simulink library "WECSim_Lib_PTOs"  (R2020b)
settings: Solver=VariableStepAuto  StartTime=0.0  StopTime=10.0  RelTol=1e-3
undefined symbols (not defined in the file or in its folder): constraint, pto, simu, X, Y, Z
libraries: nesl_utility x71, sm_lib x46, WECSim_Lib_Body_Elements x1
(part 1 of 3)
settings Model: Creator=kmruehl  LastModifiedBy=akeeste

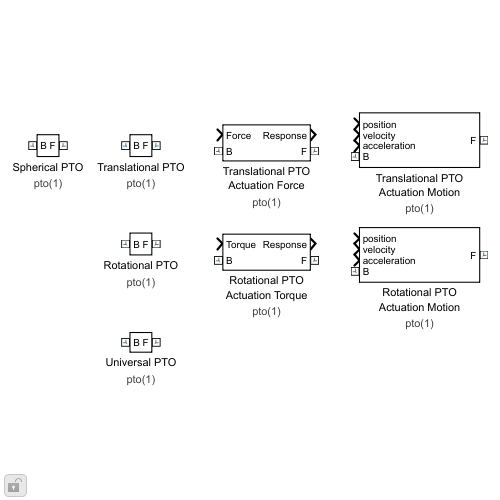
[thumbnail: Simulink's stored preview of the top-level diagram]
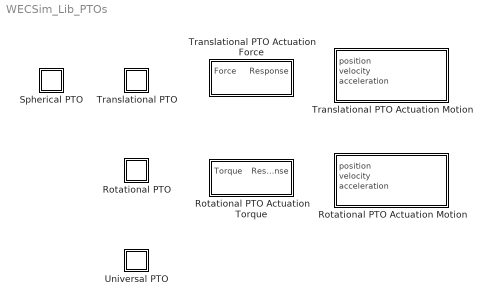
== system WECSim_Lib_PTOs ==
  Rotational PTO : Subsystem  mask(PTO){pto=pto(1)}
      mask prompts: pto "PTO Name:"
      mask help:
      | Constrains the follower to rotational motion relative to the base, about
      | the PTO's Y-direction and adds PTO stiffness and damping.
      |
      | The variable name input below must be 'pto(i)' where i=1,2,...
      | pto(i) must be defined in the input file with the following fields:
      |
      |     .name (required)
      |             String.
      |             PTO name. Must comply with Matlab's variable naming rules.
      |     .location (required)
      |             3x1 vector [x y z] in meters.
      |             PTO location. Default = [0 0 0]
      |     .stiffness (optional)
      |             Float.
      |             PTO linear spring stiffness. Default = 0
      |     .damping (optional)
      |             Float.
      |             PTO linear damping coefficient. Default = 0
      |     .orientation.z (optional)
      |             3x1 vector [x y z].
      |             Direction of the PTO's Z-coordinate. Default = [0 0 1]
      |     .orientation.y (optional)
      |             3x1 vector [x y z].
      |             Direction of the PTO's Y-coordinate. Default = [0 1 0]
      mask init:
      | if exist('pto','var')
      |     h=[gcb '/To Workspace'];
      |     responseName=['pto' num2str(pto.number) '_out'];
      |     set_param(h,'VariableName',responseName);
      |     h=[gcb '/Pitch PCC ' newline '(Revolute Joint)'];
      |     try % this should catch any version issue for which these parameters do not exist
      |         set_param(h,'upperLimitSpecify',pto.hardStops.upperLimitSpecify)
      |         set_param(h,'lowerLimitSpecify',pto.hardStops.lowerLimitSpecify)
      |     end
      |     if pto.extension.PositionTargetSpecify == 1
      |         set_param(h,'PositionTargetSpecify','on')
      |     else
      |         set_param(h,'PositionTargetSpecify','off')
      |     end
      | end
      | 
      | pto.checkLoc('E');
      settings: AttributesFormatString=%<pto>
      mask Help:
      | Constrains the follower to rotational motion relative to the base, about
      | the PTO's Y-direction and adds PTO stiffness and damping.
      | 
      | The variable name input below must be 'pto(i)' where i=1,2,...
      | pto(i) must be defined in the input file with the following fields:
      | 
      |     .name (required)
      |             String.
      |             PTO name. Must comply with Matlab's variable naming rules.
      |     .location (required)
      |             3x1 vector [x y z] in meters.
      |             PTO location. Default = [0 0 0]
      |     .stiffness (optional)
      |             Float.
      |             PTO linear spring stiffness. Default = 0
      |     .damping (optional)
      |             Float.
      |             PTO linear damping coefficient. Default = 0
      |     .orientation.z (optional)
      |             3x1 vector [x y z].
      |             Direction of the PTO's Z-coordinate. Default = [0 0 1]
      |     .orientation.y (optional)
      |             3x1 vector [x y z].
      |             Direction of the PTO's Y-coordinate. Default = [0 1 0]
  Rotational PTO Actuation Motion : Subsystem  mask(PTO){pto=pto(1)}
      mask prompts: pto "PTO Name:"
      mask help:
      | Constrains the follower to rotational motion relative to the base, about
      | the PTO's Y-direction and adds PTO stiffness and damping. Also enforces a
      | user-defined prescribed motion.
      |
      |
      | The variable name input below must be 'pto(i)' where i=1,2,...
      | pto(i) must be defined in the input file with the following fields:
      |
      |     .name (required)
      |             String.
      |             PTO name. Must comply with Matlab's variable naming rules.
      |     .location (required)
      |             3x1 vector [x y z] in meters.
      |             PTO location. Default = [0 0 0]
      |     .stiffness (optional)
      |             Float.
      |             PTO linear spring stiffness. Default = 0
      |     .damping (optional)
      |             Float.
      |             PTO linear damping coefficient. Default = 0
      |     .orientation.z (optional)
      |             3x1 vector [x y z].
      |             Direction of the PTO's Z-coordinate. Default = [0 0 1]
      |     .orientation.y (optional)
      |             3x1 vector [x y z].
      |             Direction of the PTO's Y-coordinate. Default = [0 1 0]
      mask init:
      | if exist('pto','var')
      |     h=[gcb '/To Workspace'];
      |     responseName=['pto' num2str(pto.number) '_out'];
      |     set_param(h,'VariableName',responseName);
      |     h=[gcb '/Pitch PCC ' newline '(Revolute Joint)'];
      |     try % this should catch any version issue for which these parameters do not exist
      |         set_param(h,'upperLimitSpecify',pto.hardStops.upperLimitSpecify)
      |         set_param(h,'lowerLimitSpecify',pto.hardStops.lowerLimitSpecify)
      |     end
      | end
      | 
      | pto.checkLoc('E');
      settings: AttributesFormatString=%<pto>
      mask Help:
      | Constrains the follower to rotational motion relative to the base, about
      | the PTO's Y-direction and adds PTO stiffness and damping. Also enforces a
      | user-defined prescribed motion.
      | 
      | 
      | The variable name input below must be 'pto(i)' where i=1,2,...
      | pto(i) must be defined in the input file with the following fields:
      | 
      |     .name (required)
      |             String.
      |             PTO name. Must comply with Matlab's variable naming rules.
      |     .location (required)
      |             3x1 vector [x y z] in meters.
      |             PTO location. Default = [0 0 0]
      |     .stiffness (optional)
      |             Float.
      |             PTO linear spring stiffness. Default = 0
      |     .damping (optional)
      |             Float.
      |             PTO linear damping coefficient. Default = 0
      |     .orientation.z (optional)
      |             3x1 vector [x y z].
      |             Direction of the PTO's Z-coordinate. Default = [0 0 1]
      |     .orientation.y (optional)
      |             3x1 vector [x y z].
      |             Direction of the PTO's Y-coordinate. Default = [0 1 0]
  Rotational PTO Actuation Torque : Subsystem  mask(PTO){pto=pto(1)}
      mask prompts: pto "PTO Name:"
      mask help:
      | Constrains the follower to rotational motion relative to the base, about
      | the PTO's Y-direction and adds PTO stiffness and damping. Also applies a
      | user-defined torque and outputs extension, velocity and acceleration.
      |
      |
      | The variable name input below must be 'pto(i)' where i=1,2,...
      | pto(i) must be defined in the input file with the following fields:
      |
      |     .name (required)
      |             String.
      |             PTO name. Must comply with Matlab's variable naming rules.
      |     .location (required)
      |             3x1 vector [x y z] in meters.
      |             PTO location. Default = [0 0 0]
      |     .stiffness (optional)
      |             Float.
      |             PTO linear spring stiffness. Default = 0
      |     .damping (optional)
      |             Float.
      |             PTO linear damping coefficient. Default = 0
      |     .orientation.z (optional)
      |             3x1 vector [x y z].
      |             Direction of the PTO's Z-coordinate. Default = [0 0 1]
      |     .orientation.y (optional)
      |             3x1 vector [x y z].
      |             Direction of the PTO's Y-coordinate. Default = [0 1 0]
      mask init: same as WECSim_Lib_PTOs/Rotational PTO
      settings: AttributesFormatString=%<pto>
      mask Help:
      | Constrains the follower to rotational motion relative to the base, about
      | the PTO's Y-direction and adds PTO stiffness and damping. Also applies a
      | user-defined torque and outputs extension, velocity and acceleration.
      | 
      | 
      | The variable name input below must be 'pto(i)' where i=1,2,...
      | pto(i) must be defined in the input file with the following fields:
      | 
      |     .name (required)
      |             String.
      |             PTO name. Must comply with Matlab's variable naming rules.
      |     .location (required)
      |             3x1 vector [x y z] in meters.
      |             PTO location. Default = [0 0 0]
      |     .stiffness (optional)
      |             Float.
      |             PTO linear spring stiffness. Default = 0
      |     .damping (optional)
      |             Float.
      |             PTO linear damping coefficient. Default = 0
      |     .orientation.z (optional)
      |             3x1 vector [x y z].
      |             Direction of the PTO's Z-coordinate. Default = [0 0 1]
      |     .orientation.y (optional)
      |             3x1 vector [x y z].
      |             Direction of the PTO's Y-coordinate. Default = [0 1 0]
  Spherical PTO : Subsystem  mask(PTOs){pto=pto(1)}
      mask prompts: pto "PTO Name:"
      mask help:
      | Constrains the follower to rotational motion relative to the base, fixing in
      | X,Y,Z but allowing rotation about each axis and adds PTO stiffness and damping.
      |
      | The variable name input below must be 'pto(i)' where i=1,2,...
      | pto(i) must be defined in the input file with the following fields:
      |
      |     .name (required)
      |             String.
      |            Constraint name. Must comply with Matlab's variable naming rules.
      |     .location (optional)
      |             3x1 vector [x y z] in meters.
      |             Constraint location. Default = [0 0 0]
      |     .stiffness (optional)
      |             Float.
      |             PTO linear spring stiffness. Default = 0
      |     .damping (optional)
      |             Float.
      |             PTO linear damping coefficient. Default = 0
      |     .orientation.z (optional)
      |             3x1 vector [x y z].
      |             Direction of the constraint's Z-coordinate. Default = [0 0 1]
      |     .orientation.y (optional)
      |             3x1 vector [x y z].
      |             Direction of the constraint's Y-coordinate. Default = [0 1 0]
      mask init:
      | if exist('pto','var')
      |     h=[gcb '/To Workspace'];
      |     responseName=['pto' num2str(pto.number) '_out'];
      |     set_param(h,'VariableName',responseName);
      |     h=[gcb '/Spherical Joint)'];
      |     try % this should catch any version issue for which these parameters do not exist
      |         set_param(h,'upperLimitSpecify',pto.hardStops.upperLimitSpecify)
      |         set_param(h,'lowerLimitSpecify',pto.hardStops.lowerLimitSpecify)
      |     end
      | end
      | if pto.extension.PositionTargetSpecify == 1
      |     set_param(h,'PositionTargetSpecify','on')
      | else
      |     set_param(h,'PositionTargetSpecify','off')
      | end
      | pto.checkLoc('W');
      settings: AttributesFormatString=%<pto>
      mask Help:
      | Constrains the follower to rotational motion relative to the base, fixing in
      | X,Y,Z but allowing rotation about each axis and adds PTO stiffness and damping.
      | 
      | The variable name input below must be 'pto(i)' where i=1,2,...
      | pto(i) must be defined in the input file with the following fields:
      | 
      |     .name (required)
      |             String.
      |            Constraint name. Must comply with Matlab's variable naming rules.
      |     .location (optional)
      |             3x1 vector [x y z] in meters.
      |             Constraint location. Default = [0 0 0]
      |     .stiffness (optional)
      |             Float.
      |             PTO linear spring stiffness. Default = 0
      |     .damping (optional)
      |             Float.
      |             PTO linear damping coefficient. Default = 0
      |     .orientation.z (optional)
      |             3x1 vector [x y z].
      |             Direction of the constraint's Z-coordinate. Default = [0 0 1]
      |     .orientation.y (optional)
      |             3x1 vector [x y z].
      |             Direction of the constraint's Y-coordinate. Default = [0 1 0]
  Translational PTO : Subsystem  mask(PTO){pto=pto(1)}
      mask prompts: pto "PTO Name:"
      mask help:
      | Constrains the follower to translational motion relative to the base, in
      | the PTO's Z-direction and adds PTO stiffness and damping.
      |
      |
      | The variable name input below must be 'pto(i)' where i=1,2,...
      | pto(i) must be defined in the input file with the following fields:
      |
      |     .name (required)
      |             String.
      |             PTO name. Must comply with Matlab's variable naming rules.
      |     .location (optional)
      |             3x1 vector [x y z] in meters.
      |             PTO location. Default = [0 0 0]
      |     .stiffness (optional)
      |             Float.
      |             PTO linear spring stiffness. Default = 0
      |     .damping (optional)
      |             Float.
      |             PTO linear damping coefficient. Default = 0
      |     .orientation.z (optional)
      |             3x1 vector [x y z].
      |             Direction of the PTO's Z-coordinate. Default = [0 0 1]
      |     .orientation.y (optional)
      |             3x1 vector [x y z].
      |             Direction of the PTO's Y-coordinate. Default = [0 1 0]
      mask init:
      | if exist('pto','var')
      |     h=[gcb '/To Workspace'];
      |     responseName=['pto' num2str(pto.number) '_out'];
      |     set_param(h,'VariableName',responseName);
      |     h=[gcb '/Translational PCC' newline '(Prismatic Joint)'];
      |     try % this should catch any version issue for which these parameters do not exist
      |         set_param(h,'upperLimitSpecify',pto.hardStops.upperLimitSpecify)
      |         set_param(h,'lowerLimitSpecify',pto.hardStops.lowerLimitSpecify)
      |     end
      |     if pto.extension.PositionTargetSpecify == 1
      |         set_param(h,'PositionTargetSpecify','on')
      |     else
      |         set_param(h,'PositionTargetSpecify','off')
      |     end
      | end
      | 
      | pto.checkLoc('W');
      settings: AttributesFormatString=%<pto>
      mask Help:
      | Constrains the follower to translational motion relative to the base, in
      | the PTO's Z-direction and adds PTO stiffness and damping.
      | 
      | 
      | The variable name input below must be 'pto(i)' where i=1,2,...
      | pto(i) must be defined in the input file with the following fields:
      | 
      |     .name (required)
      |             String.
      |             PTO name. Must comply with Matlab's variable naming rules.
      |     .location (optional)
      |             3x1 vector [x y z] in meters.
      |             PTO location. Default = [0 0 0]
      |     .stiffness (optional)
      |             Float.
      |             PTO linear spring stiffness. Default = 0
      |     .damping (optional)
      |             Float.
      |             PTO linear damping coefficient. Default = 0
      |     .orientation.z (optional)
      |             3x1 vector [x y z].
      |             Direction of the PTO's Z-coordinate. Default = [0 0 1]
      |     .orientation.y (optional)
      |             3x1 vector [x y z].
      |             Direction of the PTO's Y-coordinate. Default = [0 1 0]
  Translational PTO Actuation Force : Subsystem  mask(PTO){pto=pto(1)}
      mask prompts: pto "PTO Name:"
      mask help:
      | Constrains the follower to translational motion relative to the base, in
      | the PTO's Z-direction and adds PTO stiffness and damping. Also applies a
      | user-defined force and outputs extension, velocity, and acceleration.
      |
      |
      | The variable name input below must be 'pto(i)' where i=1,2,...
      | pto(i) must be defined in the input file with the following fields:
      |
      |     .name (required)
      |             String.
      |             PTO name. Must comply with Matlab's variable naming rules.
      |     .location (optional)
      |             3x1 vector [x y z] in meters.
      |             PTO location. Default = [0 0 0]
      |     .stifness (optional)
      |             Float.
      |             PTO linear spring stiffness. Default = 0
      |     .damping (optional)
      |             Float.
      |             PTO linear damping coefficient. Default = 0
      |     .orientation.z (optional)
      |             3x1 vector [x y z].
      |             Direction of the PTO's Z-coordinate. Default = [0 0 1]
      |     .orientation.y (optional)
      |             3x1 vector [x y z].
      |             Direction of the PTO's Y-coordinate. Default = [0 1 0]
      mask init:
      | if exist('pto','var')
      |     h=[gcb '/To Workspace'];
      |     responseName=['pto' num2str(pto.number) '_out'];
      |     set_param(h,'VariableName',responseName);
      |         h=[gcb '/Translational PCC' newline '(Prismatic Joint)'];
      |     try % this should catch any version issue for which these parameters do not exist
      |         set_param(h,'upperLimitSpecify',pto.hardStops.upperLimitSpecify)
      |         set_param(h,'lowerLimitSpecify',pto.hardStops.lowerLimitSpecify)
      |     end
      |     if pto.extension.PositionTargetSpecify == 1
      |         set_param(h,'PositionTargetSpecify','on')
      |     else
      |         set_param(h,'PositionTargetSpecify','off')
      |     end
      | end
      | 
      | pto.checkLoc('W');
      settings: AttributesFormatString=%<pto>
      mask Help:
      | Constrains the follower to translational motion relative to the base, in
      | the PTO's Z-direction and adds PTO stiffness and damping. Also applies a
      | user-defined force and outputs extension, velocity, and acceleration.
      | 
      | 
      | The variable name input below must be 'pto(i)' where i=1,2,...
      | pto(i) must be defined in the input file with the following fields:
      | 
      |     .name (required)
      |             String.
      |             PTO name. Must comply with Matlab's variable naming rules.
      |     .location (optional)
      |             3x1 vector [x y z] in meters.
      |             PTO location. Default = [0 0 0]
      |     .stifness (optional)
      |             Float.
      |             PTO linear spring stiffness. Default = 0
      |     .damping (optional)
      |             Float.
      |             PTO linear damping coefficient. Default = 0
      |     .orientation.z (optional)
      |             3x1 vector [x y z].
      |             Direction of the PTO's Z-coordinate. Default = [0 0 1]
      |     .orientation.y (optional)
      |             3x1 vector [x y z].
      |             Direction of the PTO's Y-coordinate. Default = [0 1 0]
  Translational PTO Actuation Motion : Subsystem  mask(PTO){pto=pto(1)}
      mask prompts: pto "PTO Name:"
      mask help:
      | Constrains the follower to translational motion relative to the base, in
      | the PTO's Z-direction and adds PTO stiffness and damping. Also enforces a
      | user-defined prescribed motion.
      |
      |
      | The variable name input below must be 'pto(i)' where i=1,2,...
      | pto(i) must be defined in the input file with the following fields:
      |
      |     .name (required)
      |             String.
      |             PTO name. Must comply with Matlab's variable naming rules.
      |     .location (optional)
      |             3x1 vector [x y z] in meters.
      |             PTO location. Default = [0 0 0]
      |     .stiffness (optional)
      |             Float.
      |             PTO linear spring stiffness. Default = 0
      |     .damping (optional)
      |             Float.
      |             PTO linear damping coefficient. Default = 0
      |     .orientation.z (optional)
      |             3x1 vector [x y z].
      |             Direction of the PTO's Z-coordinate. Default = [0 0 1]
      |     .orientation.y (optional)
      |             3x1 vector [x y z].
      |             Direction of the PTO's Y-coordinate. Default = [0 1 0]
      mask init:
      | if exist('pto','var')
      |     h=[gcb '/To Workspace'];
      |     responseName=['pto' num2str(pto.number) '_out'];
      |     set_param(h,'VariableName',responseName);
      |     h=[gcb '/Translational PCC' newline '(Prismatic Joint)'];
      |     try % this should catch any version issue for which these parameters do not exist
      |         set_param(h,'upperLimitSpecify',pto.hardStops.upperLimitSpecify)
      |         set_param(h,'lowerLimitSpecify',pto.hardStops.lowerLimitSpecify)
      |     end
      | end
      | 
      | pto.checkLoc('W');
      settings: AttributesFormatString=%<pto>
      mask Help:
      | Constrains the follower to translational motion relative to the base, in
      | the PTO's Z-direction and adds PTO stiffness and damping. Also enforces a
      | user-defined prescribed motion.
      | 
      | 
      | The variable name input below must be 'pto(i)' where i=1,2,...
      | pto(i) must be defined in the input file with the following fields:
      | 
      |     .name (required)
      |             String.
      |             PTO name. Must comply with Matlab's variable naming rules.
      |     .location (optional)
      |             3x1 vector [x y z] in meters.
      |             PTO location. Default = [0 0 0]
      |     .stiffness (optional)
      |             Float.
      |             PTO linear spring stiffness. Default = 0
      |     .damping (optional)
      |             Float.
      |             PTO linear damping coefficient. Default = 0
      |     .orientation.z (optional)
      |             3x1 vector [x y z].
      |             Direction of the PTO's Z-coordinate. Default = [0 0 1]
      |     .orientation.y (optional)
      |             3x1 vector [x y z].
      |             Direction of the PTO's Y-coordinate. Default = [0 1 0]
  Universal PTO : Subsystem  mask(PTOs){pto=pto(1)}
      mask prompts: pto "PTO Name:"
      mask help:
      | Constrains the follower to rotational motion relative to the base, fixing in
      | X,Y,Z but allowing rotation about each axis and adds PTO stiffness and damping.
      |
      | The variable name input below must be 'pto(i)' where i=1,2,...
      | pto(i) must be defined in the input file with the following fields:
      |
      |     .name (required)
      |             String.
      |            Constraint name. Must comply with Matlab's variable naming rules.
      |     .location (optional)
      |             3x1 vector [x y z] in meters.
      |             Constraint location. Default = [0 0 0]
      |     .stiffness (optional)
      |             Float.
      |             PTO linear spring stiffness. Default = 0
      |     .damping (optional)
      |             Float.
      |             PTO linear damping coefficient. Default = 0
      |     .orientation.z (optional)
      |             3x1 vector [x y z].
      |             Direction of the constraint's Z-coordinate. Default = [0 0 1]
      |     .orientation.y (optional)
      |             3x1 vector [x y z].
      |             Direction of the constraint's Y-coordinate. Default = [0 1 0]
      mask init:
      | if exist('pto','var')
      |     h=[gcb '/To Workspace'];
      |     responseName=['pto' num2str(pto.number) '_out'];
      |     set_param(h,'VariableName',responseName);
      |     h=[gcb '/Universal Joint'];
      |     try % this should catch any version issue for which these parameters do not exist
      |         set_param(h,'RxUpperLimitSpecify',pto.hardStops.upperLimitSpecify(1))
      |         set_param(h,'RxLowerLimitSpecify',pto.hardStops.lowerLimitSpecify(1))
      |         set_param(h,'RyUpperLimitSpecify',pto.hardStops.upperLimitSpecify(2))
      |         set_param(h,'RyLowerLimitSpecify',pto.hardStops.lowerLimitSpecify(2))
      |     end
      | end
      | if pto.extension.PositionTargetSpecify == 1
      |     set_param(h,'RxPositionTargetSpecify','on')
      |     set_param(h,'RyPositionTargetSpecify','on')
      | else
      |     set_param(h,'RxPositionTargetSpecify','off')
      |     set_param(h,'RyPositionTargetSpecify','off')
      | end
      | pto.checkLoc('W');
      settings: AttributesFormatString=%<pto>
      mask Help:
      | Constrains the follower to rotational motion relative to the base, fixing in
      | X,Y,Z but allowing rotation about each axis and adds PTO stiffness and damping.
      | 
      | The variable name input below must be 'pto(i)' where i=1,2,...
      | pto(i) must be defined in the input file with the following fields:
      | 
      |     .name (required)
      |             String.
      |            Constraint name. Must comply with Matlab's variable naming rules.
      |     .location (optional)
      |             3x1 vector [x y z] in meters.
      |             Constraint location. Default = [0 0 0]
      |     .stiffness (optional)
      |             Float.
      |             PTO linear spring stiffness. Default = 0
      |     .damping (optional)
      |             Float.
      |             PTO linear damping coefficient. Default = 0
      |     .orientation.z (optional)
      |             3x1 vector [x y z].
      |             Direction of the constraint's Z-coordinate. Default = [0 0 1]
      |     .orientation.y (optional)
      |             3x1 vector [x y z].
      |             Direction of the constraint's Y-coordinate. Default = [0 1 0]

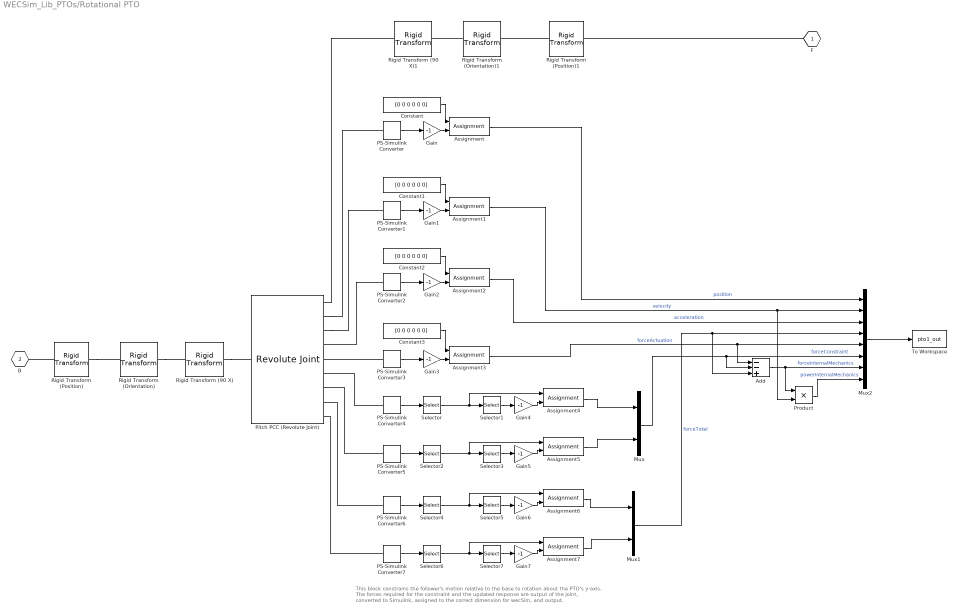
== system WECSim_Lib_PTOs/Rotational PTO ==
  note: This block constrains the follower's motion relative to the base to rotation about the PTO's y-axis. The forces required for the constraint and the updated response are output of the joint, converted to Simulink, assigned to the correct dimension for wecSim, and output.
  Add : Sum  Inputs=--+
  "Assignment " : Assignment  IndexOptions=Index vector (dialog)  Indices=5  OutputSizes=1
  Assignment1 : Assignment  IndexOptions=Index vector (dialog)  Indices=5  OutputSizes=1
  Assignment2 : Assignment  IndexOptions=Index vector (dialog)  Indices=5  OutputSizes=1
  Assignment3 : Assignment  IndexOptions=Index vector (dialog)  Indices=5  OutputSizes=1
  Assignment{4..7} (4 alike) : Assignment  DiagnosticForDimensions=Warning  IndexOptions=Index vector (dialog)  Indices=2  OutputSizes=1
  Constant{,1..3} (4 alike) : Constant  Value=[0 0 0 0 0 0]
  Gain{,1..7} (8 alike) : Gain  Gain=-1
  Mux : Mux  Inputs=2
  Mux1 : Mux  Inputs=2
  Mux2 : Mux  Inputs=8
  PS-Simulink Converter{,1..7} (8 alike) : nesl_utility/PS-Simulink Converter  PhysicalDomain=network_engine_domain  SubClassName=ps_output  LeftPortType=input  RightPortType=output  PseudoPeriodic=off  Frequencies=[]  VectorFormat=1-D array  Unit=1  AffineConversion=off
  Pitch PCC (Revolute Joint) : sm_lib/Joints/Revolute Joint  JointMode=Normal  CompositeWrenchDir=BaseOnFollower  CompositeWrenchFrame=BaseFrame  SenseConstraintForce=on  SenseConstraintTorque=on  SenseTotalForce=on  SenseTotalTorque=on  PositionTargetSpecify=off  PositionTargetPriority=High  PositionTargetValue=-pto.extension.PositionTargetValue  PositionTargetValueUnits=deg  VelocityTargetSpecify=off  VelocityTargetPriority=High  VelocityTargetValue=0  VelocityTargetValueUnits=deg/s  EquilibriumPosition=pto.equilibriumPosition  EquilibriumPositionUnits=deg  SpringStiffness=pto.stiffness  SpringStiffnessUnits=N*m/rad  DampingCoefficient=pto.damping  DampingCoefficientUnits=N*m/(rad/s)  LowerLimitSpecify=off  LowerLimitBound=pto.hardStops.lowerLimitBound  LowerLimitBoundUnits=deg  LowerLimitStiffness=pto.hardStops.lowerLimitStiffness  LowerLimitStiffnessUnits=N*m/deg  LowerLimitDamping=pto.hardStops.lowerLimitDamping  LowerLimitDampingUnits=N*m/(deg/s)  LowerLimitTransitionRegionWidth=pto.hardStops.lowerLimitTransitionRegionWidth  LowerLimitTransitionRegionWidthUnits=deg  UpperLimitSpecify=off  UpperLimitBound=pto.hardStops.upperLimitBound  UpperLimitBoundUnits=deg  UpperLimitStiffness=pto.hardStops.upperLimitStiffness  UpperLimitStiffnessUnits=N*m/deg  UpperLimitDamping=pto.hardStops.upperLimitDamping  UpperLimitDampingUnits=N*m/(deg/s)  UpperLimitTransitionRegionWidth=pto.hardStops.upperLimitTransitionRegionWidth  UpperLimitTransitionRegionWidthUnits=deg  TorqueActuationMode=NoTorque  MotionActuationMode=ComputedMotion  SensePosition=on  SenseVelocity=on  SenseAcceleration=on  SenseTorqueForce=on  SenseLowerLimitTorqueForce=off  SenseUpperLimitTorqueForce=off
  Product : Product
  Rigid Transform (Position) : sm_lib/Frames and Transforms/Rigid Transform  RotationMethod=None  FollAlignAxisA=+X  BaseAlignAxisA=+Y  FollAlignAxisB=+Y  BaseAlignAxisB=+Z  RotationStandardAxis=+Y  RotationAngle=0  RotationAngleUnits=rad  RotationArbitraryAxis=[0 1 0]  RotationSequenceAxes=FollowerAxes  RotationSequence=XYX  RotationSequenceAngles=[0 0 0]  RotationSequenceAnglesUnits=deg  RotationMatrix=[1 0 0; 0 1 0; 0 0 1]  Quaternion=[1 0 0 0]  TranslationMethod=Cartesian  TranslationCartesianOffset=pto.initial.displacement + pto.location  TranslationCartesianOffsetUnits=m  TranslationStandardAxis=+Z  TranslationStandardOffset=0  TranslationStandardOffsetUnits=m  TranslationROffset=0  TranslationROffsetUnits=m  TranslationThetaOffset=0  TranslationThetaOffsetUnits=deg  TranslationZOffset=0  TranslationZOffsetUnits=m
  Rigid Transform (Position)1 : sm_lib/Frames and Transforms/Rigid Transform  RotationMethod=None  FollAlignAxisA=+X  BaseAlignAxisA=+Y  FollAlignAxisB=+Y  BaseAlignAxisB=+Z  RotationStandardAxis=+Y  RotationAngle=0  RotationAngleUnits=rad  RotationArbitraryAxis=[0 1 0]  RotationSequenceAxes=FollowerAxes  RotationSequence=XYX  RotationSequenceAngles=[0 0 0]  RotationSequenceAnglesUnits=deg  RotationMatrix=[1 0 0; 0 1 0; 0 0 1]  Quaternion=[1 0 0 0]  TranslationMethod=Cartesian  TranslationCartesianOffset=pto.initial.displacement + pto.location  TranslationCartesianOffsetUnits=m  TranslationStandardAxis=+Z  TranslationStandardOffset=0  TranslationStandardOffsetUnits=m  TranslationROffset=0  TranslationROffsetUnits=m  TranslationThetaOffset=0  TranslationThetaOffsetUnits=deg  TranslationZOffset=0  TranslationZOffsetUnits=m
  Rigid Transform (90 X) : sm_lib/Frames and Transforms/Rigid Transform  RotationMethod=StandardAxis  FollAlignAxisA=+X  BaseAlignAxisA=+Y  FollAlignAxisB=+Y  BaseAlignAxisB=+Z  RotationStandardAxis=+X  RotationAngle=90  RotationAngleUnits=deg  RotationArbitraryAxis=[0 1 0]  RotationSequenceAxes=FollowerAxes  RotationSequence=XYX  RotationSequenceAngles=[0 0 0]  RotationSequenceAnglesUnits=deg  RotationMatrix=[1 0 0; 0 1 0; 0 0 1]  Quaternion=[1 0 0 0]  TranslationMethod=None  TranslationCartesianOffset=0  TranslationCartesianOffsetUnits=m  TranslationStandardAxis=+Z  TranslationStandardOffset=0  TranslationStandardOffsetUnits=m  TranslationROffset=0  TranslationROffsetUnits=m  TranslationThetaOffset=0  TranslationThetaOffsetUnits=deg  TranslationZOffset=0  TranslationZOffsetUnits=m
  Rigid Transform (90 X)1 : sm_lib/Frames and Transforms/Rigid Transform  RotationMethod=StandardAxis  FollAlignAxisA=+X  BaseAlignAxisA=+Y  FollAlignAxisB=+Y  BaseAlignAxisB=+Z  RotationStandardAxis=+X  RotationAngle=90  RotationAngleUnits=deg  RotationArbitraryAxis=[0 1 0]  RotationSequenceAxes=FollowerAxes  RotationSequence=XYX  RotationSequenceAngles=[0 0 0]  RotationSequenceAnglesUnits=deg  RotationMatrix=[1 0 0; 0 1 0; 0 0 1]  Quaternion=[1 0 0 0]  TranslationMethod=None  TranslationCartesianOffset=0  TranslationCartesianOffsetUnits=m  TranslationStandardAxis=+Z  TranslationStandardOffset=0  TranslationStandardOffsetUnits=m  TranslationROffset=0  TranslationROffsetUnits=m  TranslationThetaOffset=0  TranslationThetaOffsetUnits=deg  TranslationZOffset=0  TranslationZOffsetUnits=m
  Rigid Transform (Orientation) : sm_lib/Frames and Transforms/Rigid Transform  RotationMethod=RotationMatrix  FollAlignAxisA=+X  BaseAlignAxisA=+Y  FollAlignAxisB=+Y  BaseAlignAxisB=+Z  RotationStandardAxis=+Y  RotationAngle=0  RotationAngleUnits=rad  RotationArbitraryAxis=[0 1 0]  RotationSequenceAxes=FollowerAxes  RotationSequence=XYX  RotationSequenceAngles=[0 0 0]  RotationSequenceAnglesUnits=deg  RotationMatrix=pto.orientation.rotationMatrix  Quaternion=[1 0 0 0]  TranslationMethod=None  TranslationCartesianOffset=0  TranslationCartesianOffsetUnits=m  TranslationStandardAxis=+Z  TranslationStandardOffset=0  TranslationStandardOffsetUnits=m  TranslationROffset=0  TranslationROffsetUnits=m  TranslationThetaOffset=0  TranslationThetaOffsetUnits=deg  TranslationZOffset=0  TranslationZOffsetUnits=m
  Rigid Transform (Orientation)1 : sm_lib/Frames and Transforms/Rigid Transform  RotationMethod=RotationMatrix  FollAlignAxisA=+X  BaseAlignAxisA=+Y  FollAlignAxisB=+Y  BaseAlignAxisB=+Z  RotationStandardAxis=+Y  RotationAngle=0  RotationAngleUnits=rad  RotationArbitraryAxis=[0 1 0]  RotationSequenceAxes=FollowerAxes  RotationSequence=XYX  RotationSequenceAngles=[0 0 0]  RotationSequenceAnglesUnits=deg  RotationMatrix=pto.orientation.rotationMatrix  Quaternion=[1 0 0 0]  TranslationMethod=None  TranslationCartesianOffset=0  TranslationCartesianOffsetUnits=m  TranslationStandardAxis=+Z  TranslationStandardOffset=0  TranslationStandardOffsetUnits=m  TranslationROffset=0  TranslationROffsetUnits=m  TranslationThetaOffset=0  TranslationThetaOffsetUnits=deg  TranslationZOffset=0  TranslationZOffsetUnits=m
  Selector{,2,4,6} (4 alike) : Selector  InputPortWidth=3  IndexOptions=Index vector (dialog)  Indices=[1 3 2]  OutputSizes=1
  Selector{1,3,5,7} (4 alike) : Selector  InputPortWidth=3  IndexOptions=Index vector (dialog)  Indices=[2]  OutputSizes=1
  To Workspace : ToWorkspace  VariableName=pto1_out  SaveFormat=Structure With Time  SampleTime=simu.dtOut
  F : PMIOPort  Side=Right
  B : PMIOPort  Port=2  Side=Left
  wires:
  Assignment3/1 -> Add/1, Mux2/5  "forceActuation"
  Assignment2/1 -> Mux2/3  "acceleration"
  PS-Simulink Converter3/1 -> Gain3/1
  Gain3/1 -> Assignment3/2
  Constant3/1 -> Assignment3/1
  Gain2/1 -> Assignment2/2
  Constant2/1 -> Assignment2/1
  PS-Simulink Converter2/1 -> Gain2/1
  PS-Simulink Converter1/1 -> Gain1/1
  Gain1/1 -> Assignment1/2
  Constant1/1 -> Assignment1/1
  "Assignment "/1 -> Mux2/1  "position"
  Gain/1 -> "Assignment "/2
  PS-Simulink Converter/1 -> Gain/1
  Constant/1 -> "Assignment "/1
  Assignment6/1 -> Mux1/1
  Assignment7/1 -> Mux1/2
  PS-Simulink Converter7/1 -> Selector6/1
  PS-Simulink Converter6/1 -> Selector4/1
  Gain6/1 -> Assignment6/2
  Selector5/1 -> Gain6/1
  Selector4/1 -> Assignment6/1, Selector5/1
  Gain7/1 -> Assignment7/2
  Selector7/1 -> Gain7/1
  Selector6/1 -> Assignment7/1, Selector7/1
  Mux2/1 -> To Workspace/1
  PS-Simulink Converter4/1 -> Selector/1
  PS-Simulink Converter5/1 -> Selector2/1
  Assignment4/1 -> Mux/1
  Assignment5/1 -> Mux/2
  Gain4/1 -> Assignment4/2
  Selector1/1 -> Gain4/1
  Selector/1 -> Selector1/1, Assignment4/1
  Gain5/1 -> Assignment5/2
  Selector3/1 -> Gain5/1
  Selector2/1 -> Selector3/1, Assignment5/1
  Product/1 -> Mux2/8  "powerInternalMechanics"
  Assignment1/1 -> Product/2, Mux2/2  "velocity"
  Add/1 -> Mux2/7, Product/1  "forceInternalMechanics"
  Mux/1 -> Mux2/6, Add/2  "forceConstraint"
  Mux1/1 -> Add/3, Mux2/4  "forceTotal"
  connections:
  Rigid Transform (Position)/RConn1 -- Rigid Transform (Orientation)/LConn1
  Rigid Transform (Orientation)1/RConn1 -- Rigid Transform (90 X)1/LConn1
  Rigid Transform (Orientation)/RConn1 -- Rigid Transform (90 X)/LConn1
  Rigid Transform (Position)1/RConn1 -- Rigid Transform (Orientation)1/LConn1
  Rigid Transform (90 X)/RConn1 -- Pitch PCC (Revolute Joint)/LConn1
  F/RConn1 -- Rigid Transform (Position)1/LConn1
  Rigid Transform (90 X)1/RConn1 -- Pitch PCC (Revolute Joint)/RConn1
  PS-Simulink Converter3/LConn1 -- Pitch PCC (Revolute Joint)/RConn5
  PS-Simulink Converter2/LConn1 -- Pitch PCC (Revolute Joint)/RConn4
  Pitch PCC (Revolute Joint)/RConn3 -- PS-Simulink Converter1/LConn1
  Pitch PCC (Revolute Joint)/RConn2 -- PS-Simulink Converter/LConn1
  PS-Simulink Converter4/LConn1 -- Pitch PCC (Revolute Joint)/RConn6
  PS-Simulink Converter5/LConn1 -- Pitch PCC (Revolute Joint)/RConn7
  PS-Simulink Converter6/LConn1 -- Pitch PCC (Revolute Joint)/RConn8
  PS-Simulink Converter7/LConn1 -- Pitch PCC (Revolute Joint)/RConn9
  Rigid Transform (Position)/LConn1 -- B/RConn1

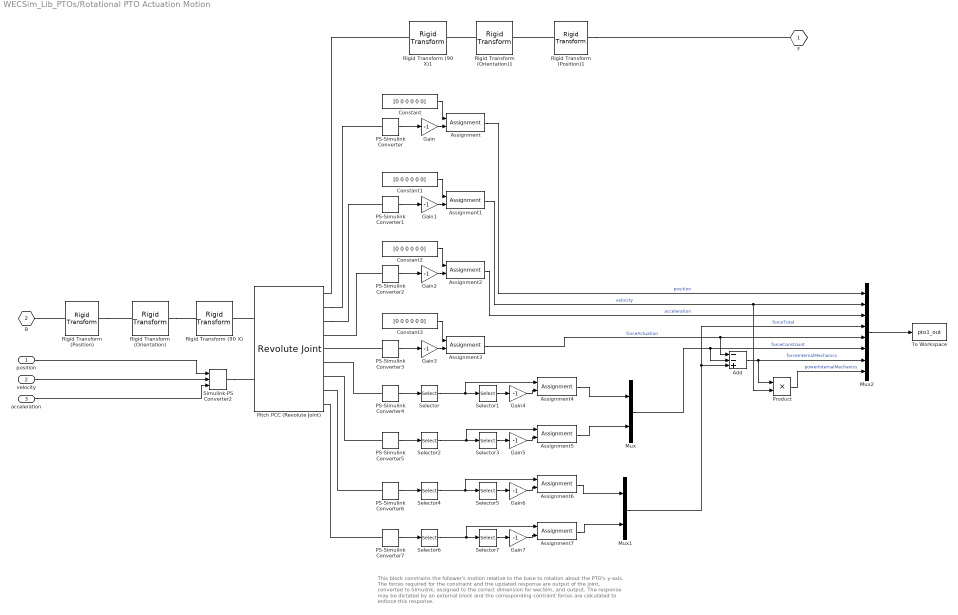
== system WECSim_Lib_PTOs/Rotational PTO Actuation Motion ==
  note: This block constrains the follower's motion relative to the base to rotation about the PTO's y-axis. The forces required for the constraint and the updated response are output of the joint, converted to Simulink, assigned to the correct dimension for wecSim, and output.
      |
      | The response may be dictated by an external block and the corresponding contraint forces are calculated to enforce this response.
  position : Inport
  velocity : Inport  Port=2
  acceleration : Inport  Port=3
  Add : Sum  Inputs=--+
  "Assignment " : Assignment  IndexOptions=Index vector (dialog)  Indices=5  OutputSizes=1
  Assignment1 : Assignment  IndexOptions=Index vector (dialog)  Indices=5  OutputSizes=1
  Assignment2 : Assignment  IndexOptions=Index vector (dialog)  Indices=5  OutputSizes=1
  Assignment3 : Assignment  IndexOptions=Index vector (dialog)  Indices=5  OutputSizes=1
  Assignment{4..7} (4 alike) : Assignment  DiagnosticForDimensions=Warning  IndexOptions=Index vector (dialog)  Indices=2  OutputSizes=1
  Constant{,1..3} (4 alike) : Constant  Value=[0 0 0 0 0 0]
  Gain{,1..7} (8 alike) : Gain  Gain=-1
  Mux : Mux  Inputs=2
  Mux1 : Mux  Inputs=2
  Mux2 : Mux  Inputs=8
  PS-Simulink Converter{,1..7} (8 alike) : nesl_utility/PS-Simulink Converter  PhysicalDomain=network_engine_domain  SubClassName=ps_output  LeftPortType=input  RightPortType=output  PseudoPeriodic=off  Frequencies=[]  VectorFormat=1-D array  Unit=1  AffineConversion=off
  Pitch PCC (Revolute Joint) : sm_lib/Joints/Revolute Joint  JointMode=Normal  CompositeWrenchDir=BaseOnFollower  CompositeWrenchFrame=BaseFrame  SenseConstraintForce=on  SenseConstraintTorque=on  SenseTotalForce=on  SenseTotalTorque=on  PositionTargetSpecify=off  PositionTargetPriority=High  PositionTargetValue=0  PositionTargetValueUnits=deg  VelocityTargetSpecify=off  VelocityTargetPriority=High  VelocityTargetValue=0  VelocityTargetValueUnits=deg/s  EquilibriumPosition=pto.equilibriumPosition  EquilibriumPositionUnits=deg  SpringStiffness=pto.stiffness  SpringStiffnessUnits=N*m/rad  DampingCoefficient=pto.damping  DampingCoefficientUnits=N*m/(rad/s)  LowerLimitSpecify=off  LowerLimitBound=pto.hardStops.lowerLimitBound  LowerLimitBoundUnits=deg  LowerLimitStiffness=pto.hardStops.lowerLimitStiffness  LowerLimitStiffnessUnits=N*m/deg  LowerLimitDamping=pto.hardStops.lowerLimitDamping  LowerLimitDampingUnits=N*m/(deg/s)  LowerLimitTransitionRegionWidth=pto.hardStops.lowerLimitTransitionRegionWidth  LowerLimitTransitionRegionWidthUnits=deg  UpperLimitSpecify=off  UpperLimitBound=pto.hardStops.upperLimitBound  UpperLimitBoundUnits=deg  UpperLimitStiffness=pto.hardStops.upperLimitStiffness  UpperLimitStiffnessUnits=N*m/deg  UpperLimitDamping=pto.hardStops.upperLimitDamping  UpperLimitDampingUnits=N*m/(deg/s)  UpperLimitTransitionRegionWidth=pto.hardStops.upperLimitTransitionRegionWidth  UpperLimitTransitionRegionWidthUnits=deg  TorqueActuationMode=ComputedTorque  MotionActuationMode=InputMotion  SensePosition=on  SenseVelocity=on  SenseAcceleration=on  SenseTorqueForce=on  SenseLowerLimitTorqueForce=off  SenseUpperLimitTorqueForce=off
  Product : Product
  Rigid Transform (Position) : sm_lib/Frames and Transforms/Rigid Transform  RotationMethod=None  FollAlignAxisA=+X  BaseAlignAxisA=+Y  FollAlignAxisB=+Y  BaseAlignAxisB=+Z  RotationStandardAxis=+Y  RotationAngle=0  RotationAngleUnits=rad  RotationArbitraryAxis=[0 1 0]  RotationSequenceAxes=FollowerAxes  RotationSequence=XYX  RotationSequenceAngles=[0 0 0]  RotationSequenceAnglesUnits=deg  RotationMatrix=[1 0 0; 0 1 0; 0 0 1]  Quaternion=[1 0 0 0]  TranslationMethod=Cartesian  TranslationCartesianOffset=pto.initial.displacement + pto.location  TranslationCartesianOffsetUnits=m  TranslationStandardAxis=+Z  TranslationStandardOffset=0  TranslationStandardOffsetUnits=m  TranslationROffset=0  TranslationROffsetUnits=m  TranslationThetaOffset=0  TranslationThetaOffsetUnits=deg  TranslationZOffset=0  TranslationZOffsetUnits=m
  Rigid Transform (Position)1 : sm_lib/Frames and Transforms/Rigid Transform  RotationMethod=None  FollAlignAxisA=+X  BaseAlignAxisA=+Y  FollAlignAxisB=+Y  BaseAlignAxisB=+Z  RotationStandardAxis=+Y  RotationAngle=0  RotationAngleUnits=rad  RotationArbitraryAxis=[0 1 0]  RotationSequenceAxes=FollowerAxes  RotationSequence=XYX  RotationSequenceAngles=[0 0 0]  RotationSequenceAnglesUnits=deg  RotationMatrix=[1 0 0; 0 1 0; 0 0 1]  Quaternion=[1 0 0 0]  TranslationMethod=Cartesian  TranslationCartesianOffset=pto.initial.displacement + pto.location  TranslationCartesianOffsetUnits=m  TranslationStandardAxis=+Z  TranslationStandardOffset=0  TranslationStandardOffsetUnits=m  TranslationROffset=0  TranslationROffsetUnits=m  TranslationThetaOffset=0  TranslationThetaOffsetUnits=deg  TranslationZOffset=0  TranslationZOffsetUnits=m
  Rigid Transform (90 X) : sm_lib/Frames and Transforms/Rigid Transform  RotationMethod=StandardAxis  FollAlignAxisA=+X  BaseAlignAxisA=+Y  FollAlignAxisB=+Y  BaseAlignAxisB=+Z  RotationStandardAxis=+X  RotationAngle=90  RotationAngleUnits=deg  RotationArbitraryAxis=[0 1 0]  RotationSequenceAxes=FollowerAxes  RotationSequence=XYX  RotationSequenceAngles=[0 0 0]  RotationSequenceAnglesUnits=deg  RotationMatrix=[1 0 0; 0 1 0; 0 0 1]  Quaternion=[1 0 0 0]  TranslationMethod=None  TranslationCartesianOffset=constraint.location  TranslationCartesianOffsetUnits=m  TranslationStandardAxis=+Z  TranslationStandardOffset=0  TranslationStandardOffsetUnits=m  TranslationROffset=0  TranslationROffsetUnits=m  TranslationThetaOffset=0  TranslationThetaOffsetUnits=deg  TranslationZOffset=0  TranslationZOffsetUnits=m
  Rigid Transform (90 X)1 : sm_lib/Frames and Transforms/Rigid Transform  RotationMethod=StandardAxis  FollAlignAxisA=+X  BaseAlignAxisA=+Y  FollAlignAxisB=+Y  BaseAlignAxisB=+Z  RotationStandardAxis=+X  RotationAngle=90  RotationAngleUnits=deg  RotationArbitraryAxis=[0 1 0]  RotationSequenceAxes=FollowerAxes  RotationSequence=XYX  RotationSequenceAngles=[0 0 0]  RotationSequenceAnglesUnits=deg  RotationMatrix=[1 0 0; 0 1 0; 0 0 1]  Quaternion=[1 0 0 0]  TranslationMethod=None  TranslationCartesianOffset=constraint.location  TranslationCartesianOffsetUnits=m  TranslationStandardAxis=+Z  TranslationStandardOffset=0  TranslationStandardOffsetUnits=m  TranslationROffset=0  TranslationROffsetUnits=m  TranslationThetaOffset=0  TranslationThetaOffsetUnits=deg  TranslationZOffset=0  TranslationZOffsetUnits=m
  Rigid Transform (Orientation) : sm_lib/Frames and Transforms/Rigid Transform  RotationMethod=RotationMatrix  FollAlignAxisA=+X  BaseAlignAxisA=+Y  FollAlignAxisB=+Y  BaseAlignAxisB=+Z  RotationStandardAxis=+Y  RotationAngle=0  RotationAngleUnits=rad  RotationArbitraryAxis=[0 1 0]  RotationSequenceAxes=FollowerAxes  RotationSequence=XYX  RotationSequenceAngles=[0 0 0]  RotationSequenceAnglesUnits=deg  RotationMatrix=pto.orientation.rotationMatrix  Quaternion=[1 0 0 0]  TranslationMethod=None  TranslationCartesianOffset=constraint.location  TranslationCartesianOffsetUnits=m  TranslationStandardAxis=+Z  TranslationStandardOffset=0  TranslationStandardOffsetUnits=m  TranslationROffset=0  TranslationROffsetUnits=m  TranslationThetaOffset=0  TranslationThetaOffsetUnits=deg  TranslationZOffset=0  TranslationZOffsetUnits=m
  Rigid Transform (Orientation)1 : sm_lib/Frames and Transforms/Rigid Transform  RotationMethod=RotationMatrix  FollAlignAxisA=+X  BaseAlignAxisA=+Y  FollAlignAxisB=+Y  BaseAlignAxisB=+Z  RotationStandardAxis=+Y  RotationAngle=0  RotationAngleUnits=rad  RotationArbitraryAxis=[0 1 0]  RotationSequenceAxes=FollowerAxes  RotationSequence=XYX  RotationSequenceAngles=[0 0 0]  RotationSequenceAnglesUnits=deg  RotationMatrix=pto.orientation.rotationMatrix  Quaternion=[1 0 0 0]  TranslationMethod=None  TranslationCartesianOffset=constraint.location  TranslationCartesianOffsetUnits=m  TranslationStandardAxis=+Z  TranslationStandardOffset=0  TranslationStandardOffsetUnits=m  TranslationROffset=0  TranslationROffsetUnits=m  TranslationThetaOffset=0  TranslationThetaOffsetUnits=deg  TranslationZOffset=0  TranslationZOffsetUnits=m
  Selector{,2,4,6} (4 alike) : Selector  InputPortWidth=3  IndexOptions=Index vector (dialog)  Indices=[1 3 2]  OutputSizes=1
  Selector{1,3,5,7} (4 alike) : Selector  InputPortWidth=3  IndexOptions=Index vector (dialog)  Indices=[2]  OutputSizes=1
  Simulink-PS Converter2 : nesl_utility/Simulink-PS Converter  PhysicalDomain=network_engine_domain  SubClassName=ps_input  LeftPortType=input  RightPortType=output  PseudoPeriodic=off  Frequencies=[]  NoiseDistribution=none  NoiseParameters=[]  Unit=1  AffineConversion=off  FilteringAndDerivatives=provide  SimscapeFilterOrder=2  InputFilterTimeConstant=0.001  UdotUserProvided=2
  To Workspace : ToWorkspace  VariableName=pto1_out  SaveFormat=Structure With Time  SampleTime=simu.dtOut
  F : PMIOPort  Side=Right
  B : PMIOPort  Port=2  Side=Left
  wires:
  position/1 -> Simulink-PS Converter2/1
  velocity/1 -> Simulink-PS Converter2/2
  acceleration/1 -> Simulink-PS Converter2/3
  PS-Simulink Converter3/1 -> Gain3/1
  Gain3/1 -> Assignment3/2
  Constant3/1 -> Assignment3/1
  Gain2/1 -> Assignment2/2
  Constant2/1 -> Assignment2/1
  PS-Simulink Converter2/1 -> Gain2/1
  PS-Simulink Converter1/1 -> Gain1/1
  Gain1/1 -> Assignment1/2
  Constant1/1 -> Assignment1/1
  Gain/1 -> "Assignment "/2
  PS-Simulink Converter/1 -> Gain/1
  Constant/1 -> "Assignment "/1
  Assignment6/1 -> Mux1/1
  Assignment7/1 -> Mux1/2
  PS-Simulink Converter7/1 -> Selector6/1
  PS-Simulink Converter6/1 -> Selector4/1
  Gain6/1 -> Assignment6/2
  Selector5/1 -> Gain6/1
  Selector4/1 -> Assignment6/1, Selector5/1
  Gain7/1 -> Assignment7/2
  Selector7/1 -> Gain7/1
  Selector6/1 -> Assignment7/1, Selector7/1
  Mux2/1 -> To Workspace/1
  PS-Simulink Converter4/1 -> Selector/1
  PS-Simulink Converter5/1 -> Selector2/1
  Assignment4/1 -> Mux/1
  Assignment5/1 -> Mux/2
  Gain4/1 -> Assignment4/2
  Selector1/1 -> Gain4/1
  Selector/1 -> Selector1/1, Assignment4/1
  Gain5/1 -> Assignment5/2
  Selector3/1 -> Gain5/1
  Selector2/1 -> Selector3/1, Assignment5/1
  Assignment2/1 -> Mux2/3  "acceleration"
  "Assignment "/1 -> Mux2/1  "position"
  Assignment1/1 -> Product/2, Mux2/2  "velocity"
  Add/1 -> Mux2/7, Product/1  "forceInternalMechanics"
  Mux1/1 -> Add/3, Mux2/4  "forceTotal"
  Assignment3/1 -> Add/1, Mux2/5  "forceActuation"
  Mux/1 -> Add/2, Mux2/6  "forceConstraint"
  Product/1 -> Mux2/8  "powerInternalMechanics"
  connections:
  Rigid Transform (Position)/RConn1 -- Rigid Transform (Orientation)/LConn1
  Rigid Transform (Orientation)/RConn1 -- Rigid Transform (90 X)/LConn1
  Rigid Transform (Orientation)1/RConn1 -- Rigid Transform (90 X)1/LConn1
  Rigid Transform (Position)1/RConn1 -- Rigid Transform (Orientation)1/LConn1
  Pitch PCC (Revolute Joint)/LConn1 -- Rigid Transform (90 X)/RConn1
  Rigid Transform (90 X)1/RConn1 -- Pitch PCC (Revolute Joint)/RConn1
  Simulink-PS Converter2/RConn1 -- Pitch PCC (Revolute Joint)/LConn2
  Rigid Transform (Position)1/LConn1 -- F/RConn1
  PS-Simulink Converter3/LConn1 -- Pitch PCC (Revolute Joint)/RConn5
  PS-Simulink Converter2/LConn1 -- Pitch PCC (Revolute Joint)/RConn4
  Pitch PCC (Revolute Joint)/RConn3 -- PS-Simulink Converter1/LConn1
  Pitch PCC (Revolute Joint)/RConn2 -- PS-Simulink Converter/LConn1
  PS-Simulink Converter4/LConn1 -- Pitch PCC (Revolute Joint)/RConn6
  PS-Simulink Converter5/LConn1 -- Pitch PCC (Revolute Joint)/RConn7
  PS-Simulink Converter6/LConn1 -- Pitch PCC (Revolute Joint)/RConn8
  PS-Simulink Converter7/LConn1 -- Pitch PCC (Revolute Joint)/RConn9
  Rigid Transform (Position)/LConn1 -- B/RConn1
